simulink model "tanque_feedforward"  (Simulink 8.3)
settings: Solver=ode45  StartTime=0.0  StopTime=600  RelTol=1e-3
settings Model: Creator=Lideq2  LastModifiedBy=marcio
settings OptimizationCC: ExpressionDepthLimit=2147483647  InitFltsAndDblsToZero=on
settings DebuggingCC: SaveWithParameterizedLinksMsg=none  MultiTaskDSMMsg=warning  MultiTaskCondExecSysMsg=none  FcnCallInpInsideContextMsg=UseLocalSettings
settings RTWCC: IncludeERTFirstTime=on
settings GRTTargetCC: TargetFcnLib=ansi_tfl_tmw.mat

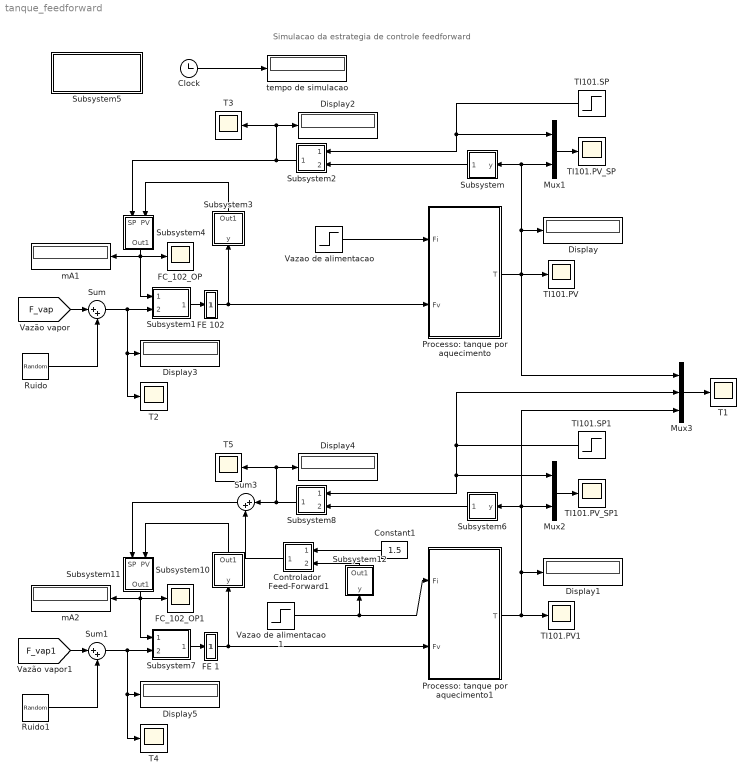
== system tanque_feedforward ==
  note: Simulacao da estrategia de controle feedforward
  Clock : Clock
  Constant1 : Constant  Value=1.5
  Controlador  Feed-Forward1 : Subsystem
      mask Display:
      | disp('AX\n411')
      | 
      | plot([   -5.0000   -4.9000   -4.8000   -4.7000    -4.6000   -4.5000   -4.4000   -4.3000  -4.2000   -4.1000   -4.0000   -3.9000    -3.8000   -3.7000   -3.6000   -3.5000    -3.4000   -3.3000   -3.2000   -3.1000    -3.0000   -2.9000   -2.8000   -2.7000    -2.6000   -2.5000   -2.4000   -2.3000    -2.2000   -2.1000   -2.0000   -1.9000    -1.8000   -1.7000   -1.6000   -1.5000    -1.4000   -1.3000   -1.2000   -1.1000    -1.0000   -0.9000   -0.8000   -0.7000    -0.6000   -0.5000   -0.4000   -0.3000    -0.2000   -0.1000         0    0.1000     0.2000    0.3000    0.4000    0.5000     0.6000    0.7000    0.8000    0.9000     1.0000    1.1000    1.2000    1.3000     1.4000    1.5000    1.6000    1.7000     1.8000    1.9000    2.0000    2.1000     2.2000    2.3000    2.4000    2.5000     2.6000    2.7000    2.8000    2.9000     3.0000    3.1000    3.2000    3.3000     3.4000    3.5000    3.6000    3.7000     3.8000    3.9000    4.0000    4.1000     4.2000    4.3000    4.4000    4.5000     4.6000    4.7000    4.8000    4.9000     5.0000], [0    0.9950    1.4000    1.7059     1.9596    2.1794    2.3749    2.5515    2.7129    2.8618    3.0000    3.1289    3.2496    3.3630    3.4699    3.5707     3.6661    3.7563    3.8419    3.9230    4.0000    4.0731    4.1425    4.2083    4.2708    4.3301    4.3863    4.4396    4.4900    4.5376    4.5826    4.6249    4.6648    4.7021    4.7371    4.7697    4.8000    4.8280    4.8539    4.8775     4.8990    4.9183    4.9356    4.9508    4.9639    4.9749    4.9840    4.9910    4.9960    4.9990    5.0000    4.9990    4.9960    4.9910    4.9840    4.9749    4.9639    4.9508    4.9356    4.9183    4.8990    4.8775    4.8539    4.8280    4.8000    4.7697    4.7371    4.7021    4.6648    4.6249    4.5826    4.5376    4.4900    4.4396    4.3863    4.3301    4.2708    4.2083    4.1425    4.0731    4.0000    3.9230    3.8419    3.7563    3.6661    3.5707    3.4699    3.3630    3.2496    3.1289    3.0000    2.8618    2.7129    2.5515    2.3749    2.1794     1.9596    1.7059    1.4000    0.9950         0], [   -5.0000   -4.9000   -4.8000   -4.7000    -4.6000   -4.5000   -4.4000   -4.3000  -4.2000   -4.1000   -4.0000   -3.9000    -3.8000   -3.7000   -3.6000   -3.5000    -3.4000   -3.3000   -3.2000   -3.1000    -3.0000   -2.9000   -2.8000   -2.7000    -2.6000   -2.5000   -2.4000   -2.3000    -2.2000   -2.1000   -2.0000   -1.9000    -1.8000   -1.7000   -1.6000   -1.5000    -1.4000   -1.3000   -1.2000   -1.1000    -1.0000   -0.9000   -0.8000   -0.7000    -0.6000   -0.5000   -0.4000   -0.3000    -0.2000   -0.1000         0    0.1000     0.2000    0.3000    0.4000    0.5000     0.6000    0.7000    0.8000    0.9000     1.0000    1.1000    1.2000    1.3000     1.4000    1.5000    1.6000    1.7000     1.8000    1.9000    2.0000    2.1000     2.2000    2.3000    2.4000    2.5000     2.6000    2.7000    2.8000    2.9000     3.0000    3.1000    3.2000    3.3000     3.4000    3.5000    3.6000    3.7000     3.8000    3.9000    4.0000    4.1000     4.2000    4.3000    4.4000    4.5000     4.6000    4.7000    4.8000    4.9000     5.0000], -[0    0.9950    1.4000    1.7059     1.9596    2.1794    2.3749    2.5515    2.7129    2.8618    3.0000    3.1289    3.2496    3.3630    3.4699    3.5707     3.6661    3.7563    3.8419    3.9230    4.0000    4.0731    4.1425    4.2083    4.2708    4.3301    4.3863    4.4396    4.4900    4.5376    4.5826    4.6249    4.6648    4.7021    4.7371    4.7697    4.8000    4.8280    4.8539    4.8775     4.8990    4.9183    4.9356    4.9508    4.9639    4.9749    4.9840    4.9910    4.9960    4.9990    5.0000    4.9990    4.9960    4.9910    4.9840    4.9749    4.9639    4.9508    4.9356    4.9183    4.8990    4.8775    4.8539    4.8280    4.8000    4.7697    4.7371    4.7021    4.6648    4.6249    4.5826    4.5376    4.4900    4.4396    4.3863    4.3301    4.2708    4.2083    4.1425    4.0731    4.0000    3.9230    3.8419    3.7563    3.6661    3.5707    3.4699    3.3630    3.2496    3.1289    3.0000    2.8618    2.7129    2.5515    2.3749    2.1794     1.9596    1.7059    1.4000    0.9950         0])
  Display{,1..5} (6 alike) : Display
  FC_102_OP : Scope
      settings: SaveName=FC_102_OP
  FC_102_OP1 : Scope
      settings: SaveName=FC_102_OP1
  FE 1 : Subsystem
      mask Display: plot(-1*ones(1,21),[-2:0.2:2],zeros(1,11),[-1:0.2:1],1*ones(1,21),[-2:0.2:2])
  FE 102 : Subsystem
      mask Display: plot(-1*ones(1,21),[-2:0.2:2],zeros(1,11),[-1:0.2:1],1*ones(1,21),[-2:0.2:2])
  Mux1 : Mux  Inputs=2
  Mux2 : Mux  Inputs=2
  Mux3 : Mux  Inputs=3
  Processo: tanque por aquecimento : Subsystem  mask(Teste){Fi=1.5, Fv=0.4, T=57}
      mask prompts: Fi "Estado estacionário da vazão de alimentação do tanque [=] t/min"; Fv "Estado estacionário da vazão de vapor do tanque [=] t/min"; T "Temperatura de saída do tanque"
      mask help: Testando descrição
      mask init:
      | x = -1:.1:1;
      | y1 =  x;
      | y2 = -x;
      | 
      | x1 = zeros(1,3);
      | y3 = [0 1 7];
      | 
      | y4 = -1:.1:1;
      | r = sqrt(2);
      | x2 = sqrt(r^2-y4.^2);
      | x3 = -sqrt(r^2-y4.^2);
      | 
      | xs = -sqrt(2)-.5:0.1:sqrt(2)+.5;
      | ys = sin(10000*xs)/3-sqrt(2)-.3;
      | 
      | y1t = y1 + 3;
      | y2t = y2 + 3;
      | 
      | y4t = 2:.1:4;
      | x2t =  sqrt(r^2-(y4t-3).^2);
      | x3t = -sqrt(r^2-(y4t-3).^2);
      mask Help: TESTANDO HELP
      mask Display:
      | plot(x,y1,x,y2,x1,y3,x2,y4,x3,y4,xs,ys)
      | plot(x,y1t,x,y2t,x2t,y4t,x3t,y4t)
      | plot(sqrt(2)+0.5,0,-sqrt(2)-0.5,0)
  Processo: tanque por aquecimento1 : Subsystem  mask(Teste){Fi=1.5, Fv=0.4, T=57}
      mask prompts: Fi "Estado estacionário da vazão de alimentação do tanque [=] t/min"; Fv "Estado estacionário da vazão de vapor do tanque [=] t/min"; T "Temperatura de saída do tanque"
      mask help: Testando descrição
      mask init: same as tanque_feedforward/Processo: tanque por aquecimento
      mask Help: TESTANDO HELP
      mask Display:
      | plot(x,y1,x,y2,x1,y3,x2,y4,x3,y4,xs,ys)
      | plot(x,y1t,x,y2t,x2t,y4t,x3t,y4t)
      | plot(sqrt(2)+0.5,0,-sqrt(2)-0.5,0)
  Ruido : RandomNumber  Variance=0.001  SampleTime=0
  Ruido1 : RandomNumber  Variance=0.001  SampleTime=0
  Subsystem : Subsystem  mask(Transmissor){ymax=100, ymin=0}
      mask prompts: ymax "Valor máximo da variavel"; ymin "Valor minimo da variavel"
      mask init:
      | x = -1:.1:1;
      | r = 1;
      | y1 = sqrt(r^2 - x.^2);
      | y2 = -sqrt(r^2 - x.^2);
      mask Display:
      | disp('TT')
      | plot(x,y1,x,y2)
  Subsystem1 : Subsystem  mask{Fmax=0.8, Fmin=0, talv=0.05}
      mask prompts: Fmax "Vazão máxima da valvula"; Fmin "Vazão minima da valvula"; talv "Dinâmica da valvula"
      mask init:
      | x= -1:.1:1;
      | 
      | y1=x;
      | y2=-x;
      | 
      | x1=[1,1];
      | y3=[1,-1];
      | x2=[-1,-1];
      | 
      | x3=[0,0,0];
      | y4=[0,1,2];
      | 
      | r=0.8;
      | x6= -r:.1:r;
      | y6 = sqrt(r^2-x6.^2)+2;
      | 
      | x5= [-r,r];
      | y5=[2,2];
      mask Display:
      | plot(x,y1,x,y2,x1,y3,x2,y3,x3,y4,x5,y5)
      | plot(x6,y6)
  Subsystem10 : Subsystem  mask(Transmissor){ymax=0.4*2, ymin=0}
      mask prompts: ymax "Valor máximo da variavel"; ymin "Valor minimo da variavel"
      mask init:
      | x = -1:.1:1;
      | r = 1;
      | y1 = sqrt(r^2 - x.^2);
      | y2 = -sqrt(r^2 - x.^2);
      mask Display:
      | disp('FT')
      | plot(x,y1,x,y2)
  Subsystem11 : Subsystem  mask(Controlador){AC=1, kc=3, tal_i=0.05, tal_d=0, BIAS=50, MODO=1}
      mask prompts: AC "Ação do controlador"; kc "Ganho do controlador"; tal_i "Constante de tempo integral"; tal_d "Constante de tempo derivativa"; BIAS "Posição da valvula em manual"; MODO "Modo de controle"
      mask init:
      | x = -1:.1:1;
      | r = 1;
      | y1 = sqrt(r^2 - x.^2);
      | y2 = -sqrt(r^2 - x.^2);
      mask Display:
      | disp('FC')
      | plot(x,y1,x,y2)
  Subsystem12 : Subsystem  mask(Transmissor){ymax=1.5*2, ymin=0}
      mask prompts: ymax "Valor máximo da variavel"; ymin "Valor minimo da variavel"
      mask init:
      | x = -1:.1:1;
      | r = 1;
      | y1 = sqrt(r^2 - x.^2);
      | y2 = -sqrt(r^2 - x.^2);
      mask Display:
      | disp('FT')
      | plot(x,y1,x,y2)
  Subsystem2 : Subsystem  mask(Controlador){AC=1, kc=2.4, tal_i=4.32, tal_d=0.05, BIAS=50, MODO=1}
      mask prompts: AC "Ação do controlador"; kc "Ganho do controlador"; tal_i "Constante de tempo integral"; tal_d "Constante de tempo derivativa"; BIAS "Posição da valvula em manual"; MODO "Modo de controle"
      mask init:
      | x = -1:.1:1;
      | r = 1;
      | y1 = sqrt(r^2 - x.^2);
      | y2 = -sqrt(r^2 - x.^2);
      mask Display:
      | disp('TC')
      | plot(x,y1,x,y2)
  Subsystem3 : Subsystem  mask(Transmissor){ymax=0.4*2, ymin=0}
      mask prompts: ymax "Valor máximo da variavel"; ymin "Valor minimo da variavel"
      mask init:
      | x = -1:.1:1;
      | r = 1;
      | y1 = sqrt(r^2 - x.^2);
      | y2 = -sqrt(r^2 - x.^2);
      mask Display:
      | disp('FT')
      | plot(x,y1,x,y2)
  Subsystem4 : Subsystem  mask(Controlador){AC=1, kc=3, tal_i=0.05, tal_d=0, BIAS=50, MODO=1}
      mask prompts: AC "Ação do controlador"; kc "Ganho do controlador"; tal_i "Constante de tempo integral"; tal_d "Constante de tempo derivativa"; BIAS "Posição da valvula em manual"; MODO "Modo de controle"
      mask init:
      | x = -1:.1:1;
      | r = 1;
      | y1 = sqrt(r^2 - x.^2);
      | y2 = -sqrt(r^2 - x.^2);
      mask Display:
      | disp('FC')
      | plot(x,y1,x,y2)
  Subsystem5 : Subsystem
      settings: OpenFcn=save tanque
      mask Display: disp('Salvar \n dados')
  Subsystem6 : Subsystem  mask(Transmissor){ymax=100, ymin=0}
      mask prompts: ymax "Valor máximo da variavel"; ymin "Valor minimo da variavel"
      mask init:
      | x = -1:.1:1;
      | r = 1;
      | y1 = sqrt(r^2 - x.^2);
      | y2 = -sqrt(r^2 - x.^2);
      mask Display:
      | disp('TT')
      | plot(x,y1,x,y2)
  Subsystem7 : Subsystem  mask{Fmax=0.8, Fmin=0, talv=0.05}
      mask prompts: Fmax "Vazão máxima da valvula"; Fmin "Vazão minima da valvula"; talv "Dinâmica da valvula"
      mask init:
      | x= -1:.1:1;
      | 
      | y1=x;
      | y2=-x;
      | 
      | x1=[1,1];
      | y3=[1,-1];
      | x2=[-1,-1];
      | 
      | x3=[0,0,0];
      | y4=[0,1,2];
      | 
      | r=0.8;
      | x6= -r:.1:r;
      | y6 = sqrt(r^2-x6.^2)+2;
      | 
      | x5= [-r,r];
      | y5=[2,2];
      mask Display:
      | plot(x,y1,x,y2,x1,y3,x2,y3,x3,y4,x5,y5)
      | plot(x6,y6)
  Subsystem8 : Subsystem  mask(Controlador){AC=1, kc=2.4, tal_i=4.32, tal_d=0.05, BIAS=50, MODO=1}
      mask prompts: AC "Ação do controlador"; kc "Ganho do controlador"; tal_i "Constante de tempo integral"; tal_d "Constante de tempo derivativa"; BIAS "Posição da valvula em manual"; MODO "Modo de controle"
      mask init:
      | x = -1:.1:1;
      | r = 1;
      | y1 = sqrt(r^2 - x.^2);
      | y2 = -sqrt(r^2 - x.^2);
      mask Display:
      | disp('TC')
      | plot(x,y1,x,y2)
  Sum : Sum  Inputs=|++
  Sum1 : Sum  Inputs=|++
  Sum3 : Sum  Inputs=|++
  T{1..5} (5 alike) : Scope
      T1 settings: SaveName=ScopeData9
      T2 settings: SaveName=ScopeData2
      T3 settings: SaveName=ScopeData4
      T4 settings: SaveName=ScopeData5
      T5 settings: SaveName=ScopeData6
  TI101.PV : Scope
  TI101.PV1 : Scope
      settings: SaveName=ScopeData7
  TI101.PV_SP : Scope
  TI101.PV_SP1 : Scope
      settings: SaveName=ScopeData8
  TI101.SP : Step  Time=50  Before=57  After=57*1.1  SampleTime=0
  TI101.SP1 : Step  Time=50  Before=57  After=57*1.1  SampleTime=0
  Vazao de alimentacao : Step  Time=300  Before=1.5  After=1.5*1.35  SampleTime=0
  Vazao de alimentacao1 : Step  Time=300  Before=1.5  After=1.5*1.35  SampleTime=0
  mA1 : Display
  mA2 : Display
  tempo de simulacao : Display
  wires:
  Processo: tanque por aquecimento/1(T) -> TI101.PV/1, Display/1, Subsystem/1(y), Mux1/2, Mux3/1
  Vazao de alimentacao/1 -> Processo: tanque por aquecimento/1(Fi)
  Subsystem/1(Out1) -> Subsystem2/2(PV)
  Subsystem2/1(Out1) -> Display2/1, T3/1, Subsystem4/1(SP)
  Mux1/1 -> TI101.PV_SP/1
  TI101.SP/1 -> Subsystem2/1(SP), Mux1/1
  Sum/1 -> Subsystem1/2(In2), Display3/1, T2/1
  [F_vap] -> Sum/1
  Ruido/1 -> Sum/2
  Subsystem3/1(Out1) -> Subsystem4/2(PV)
  Subsystem1/1(Out2) -> FE 102/1(In1)
  FE 102/1(Out2) -> Processo: tanque por aquecimento/2(Fv), Subsystem3/1(y)
  Subsystem4/1(Out1) -> FC_102_OP/1, mA1/1, Subsystem1/1(In1)
  Clock/1 -> tempo de simulacao/1
  Mux3/1 -> T1/1
  Processo: tanque por aquecimento1/1(T) -> Mux2/2, Subsystem6/1(y), Mux3/3, Display1/1, TI101.PV1/1
  Vazao de alimentacao1/1 -> Processo: tanque por aquecimento1/1(Fi), Subsystem12/1(y)
  Subsystem6/1(Out1) -> Subsystem8/2(PV)
  Subsystem8/1(Out1) -> Sum3/1, T5/1, Display4/1
  Mux2/1 -> TI101.PV_SP1/1
  TI101.SP1/1 -> Mux2/1, Subsystem8/1(SP), Mux3/2
  Sum1/1 -> T4/1, Display5/1, Subsystem7/2(In2)
  [F_vap1] -> Sum1/1
  Ruido1/1 -> Sum1/2
  Subsystem10/1(Out1) -> Subsystem11/2(PV)
  Subsystem7/1(Out2) -> FE 1/1(In1)
  FE 1/1(Out2) -> Subsystem10/1(y), Processo: tanque por aquecimento1/2(Fv)
  Subsystem11/1(Out1) -> Subsystem7/1(In1), mA2/1, FC_102_OP1/1
  Constant1/1 -> Controlador  Feed-Forward1/1(Set-Point do distúrbio externo)
  Sum3/1 -> Subsystem11/1(SP)
  Controlador  Feed-Forward1/1(Out1) -> Sum3/2
  Subsystem12/1(Out1) -> Controlador  Feed-Forward1/2(Sinal do distúrbio externo)

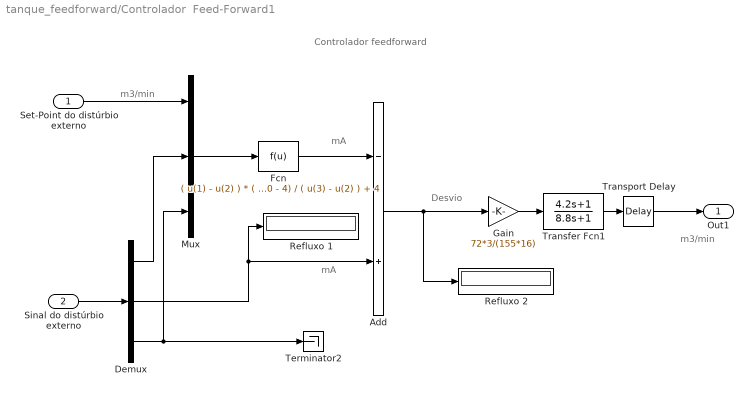
== system tanque_feedforward/Controlador  Feed-Forward1 ==
  note: m3/min
  note: Desvio
  note: mA
  note: mA
  note: m3/min
  note: Controlador feedforward
  Set-Point do distúrbio externo : Inport
  Sinal do distúrbio externo : Inport  Port=2
  Add : Sum  Inputs=-+
  Demux : Demux  Outputs=3
  Fcn : Fcn  Expr=( u(1) - u(2) ) * ( 20 - 4) / ( u(3) - u(2) ) + 4
  Gain : Gain  Gain=72*3/(155*16)
  Mux : Mux  Inputs=3
  Refluxo 1 : Display
  Refluxo 2 : Display
  Terminator2 : Terminator
  Transfer Fcn1 : TransferFcn  Numerator=[4.2 1]  Denominator=[8.8 1]
  Transport Delay : TransportDelay  DelayTime=2
  Out1 : Outport
  wires:
  Demux/1 -> Mux/2
  Demux/2 -> Refluxo 1/1, Add/2
  Transport Delay/1 -> Out1/1
  Add/1 -> Refluxo 2/1, Gain/1
  Fcn/1 -> Add/1
  Mux/1 -> Fcn/1
  Set-Point do distúrbio externo/1 -> Mux/1
  Demux/3 -> Mux/3, Terminator2/1
  Sinal do distúrbio externo/1 -> Demux/1
  Transfer Fcn1/1 -> Transport Delay/1
  Gain/1 -> Transfer Fcn1/1

== system tanque_feedforward/FE 1 ==
  note: Placa de orifício
  In1 : Inport
  Out2 : Outport
  wires:
  In1/1 -> Out2/1

== system tanque_feedforward/FE 102 ==
  note: Placa de orifício
  In1 : Inport
  Out2 : Outport
  wires:
  In1/1 -> Out2/1

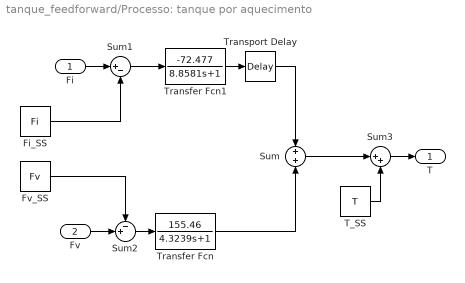
== system tanque_feedforward/Processo: tanque por aquecimento ==
  Fi : Inport
  Fv : Inport  Port=2
  Fi_SS : Constant  Value=Fi
  Fv_SS : Constant  Value=Fv
  Sum : Sum  Inputs=+|+
  Sum1 : Sum  Inputs=|+-
  Sum2 : Sum  Inputs=-+|
  Sum3 : Sum  Inputs=|++
  T_SS : Constant  Value=T
  Transfer Fcn : TransferFcn  Numerator=[155.46]  Denominator=[4.3239 1]
  Transfer Fcn1 : TransferFcn  Numerator=[-72.477]  Denominator=[8.8581 1]
  Transport Delay : TransportDelay  DelayTime=2
  T : Outport
  wires:
  Sum/1 -> Sum3/1
  T_SS/1 -> Sum3/2
  Fi_SS/1 -> Sum1/2
  Fv_SS/1 -> Sum2/1
  Fi/1 -> Sum1/1
  Sum3/1 -> T/1
  Fv/1 -> Sum2/2
  Sum1/1 -> Transfer Fcn1/1
  Sum2/1 -> Transfer Fcn/1
  Transfer Fcn1/1 -> Transport Delay/1
  Transport Delay/1 -> Sum/1
  Transfer Fcn/1 -> Sum/2

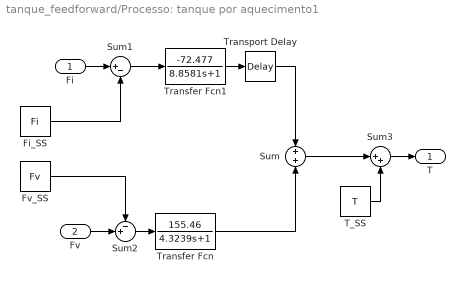
== system tanque_feedforward/Processo: tanque por aquecimento1 ==
  Fi : Inport
  Fv : Inport  Port=2
  Fi_SS : Constant  Value=Fi
  Fv_SS : Constant  Value=Fv
  Sum : Sum  Inputs=+|+
  Sum1 : Sum  Inputs=|+-
  Sum2 : Sum  Inputs=-+|
  Sum3 : Sum  Inputs=|++
  T_SS : Constant  Value=T
  Transfer Fcn : TransferFcn  Numerator=[155.46]  Denominator=[4.3239 1]
  Transfer Fcn1 : TransferFcn  Numerator=[-72.477]  Denominator=[8.8581 1]
  Transport Delay : TransportDelay  DelayTime=2
  T : Outport
  wires:
  Transfer Fcn/1 -> Sum/2
  Transport Delay/1 -> Sum/1
  Transfer Fcn1/1 -> Transport Delay/1
  Sum2/1 -> Transfer Fcn/1
  Sum1/1 -> Transfer Fcn1/1
  Fv/1 -> Sum2/2
  Sum3/1 -> T/1
  Fi/1 -> Sum1/1
  Fv_SS/1 -> Sum2/1
  Fi_SS/1 -> Sum1/2
  T_SS/1 -> Sum3/2
  Sum/1 -> Sum3/1

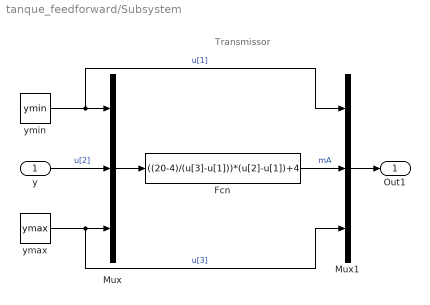
== system tanque_feedforward/Subsystem ==
  note: Transmissor
  y : Inport
  Fcn : Fcn  Expr=((20-4)/(u[3]-u[1]))*(u[2]-u[1])+4
  Mux : Mux  Inputs=3
  Mux1 : Mux  Inputs=3
  ymax : Constant  Value=ymax
  ymin : Constant  Value=ymin
  Out1 : Outport
  wires:
  ymin/1 -> Mux/1, Mux1/1  "u[1]"
  y/1 -> Mux/2  "u[2]"
  ymax/1 -> Mux/3, Mux1/3  "u[3]"
  Mux/1 -> Fcn/1
  Fcn/1 -> Mux1/2  "mA"
  Mux1/1 -> Out1/1

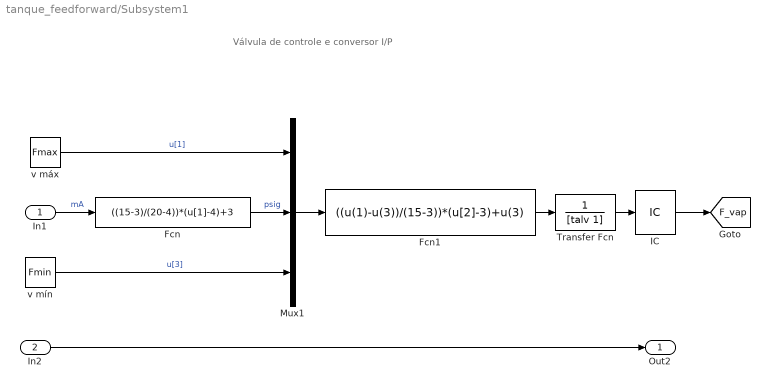
== system tanque_feedforward/Subsystem1 ==
  note: Válvula de controle e conversor I/P
  In1 : Inport
  In2 : Inport  Port=2
  Fcn : Fcn  Expr=((15-3)/(20-4))*(u[1]-4)+3
  Fcn1 : Fcn  Expr=((u(1)-u(3))/(15-3))*(u[2]-3)+u(3)
  IC : InitialCondition  Value=0.4
  Mux1 : Mux  Inputs=3
  Transfer Fcn : TransferFcn  Denominator=[talv 1]
  v máx : Constant  Value=Fmax
  v mín : Constant  Value=Fmin
  Out2 : Outport
  tag scope: F_vap=global
  wires:
  Fcn/1 -> Mux1/2  "psig"
  In1/1 -> Fcn/1  "mA"
  Mux1/1 -> Fcn1/1
  v máx/1 -> Mux1/1  "u[1]"
  v mín/1 -> Mux1/3  "u[3]"
  In2/1 -> Out2/1
  Fcn1/1 -> Transfer Fcn/1
  IC/1 -> [F_vap]
  Transfer Fcn/1 -> IC/1

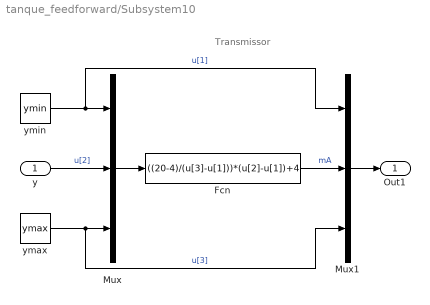
== system tanque_feedforward/Subsystem10 ==
  note: Transmissor
  y : Inport
  Fcn : Fcn  Expr=((20-4)/(u[3]-u[1]))*(u[2]-u[1])+4
  Mux : Mux  Inputs=3
  Mux1 : Mux  Inputs=3
  ymax : Constant  Value=ymax
  ymin : Constant  Value=ymin
  Out1 : Outport
  wires:
  ymin/1 -> Mux/1, Mux1/1  "u[1]"
  y/1 -> Mux/2  "u[2]"
  ymax/1 -> Mux/3, Mux1/3  "u[3]"
  Mux/1 -> Fcn/1
  Fcn/1 -> Mux1/2  "mA"
  Mux1/1 -> Out1/1

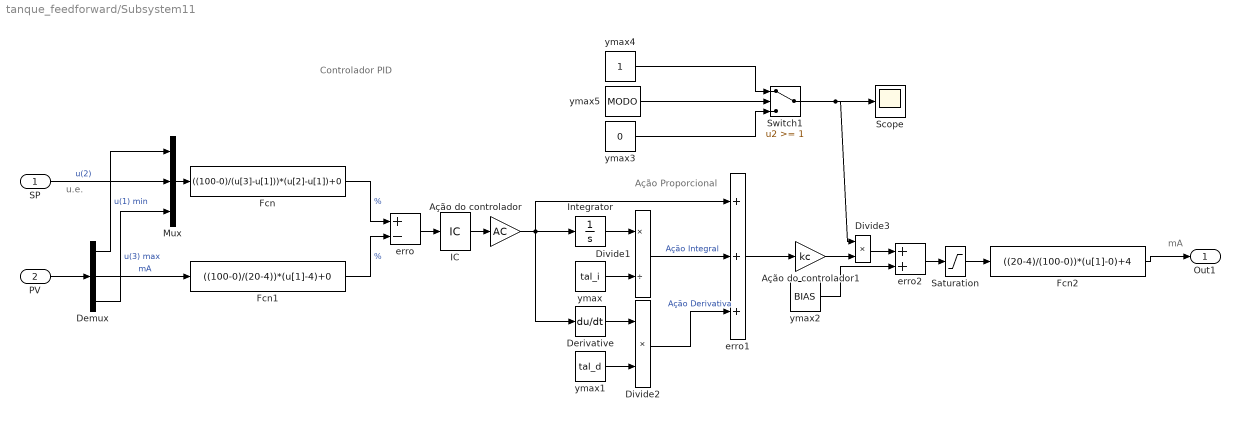
== system tanque_feedforward/Subsystem11 ==
  note: Controlador PID
  note: u.e.
  note: Ação Proporcional
  note: mA
  SP : Inport
  PV : Inport  Port=2
  Ação do controlador : Gain  Gain=AC
  Ação do controlador1 : Gain  Gain=kc
  Demux : Demux  Outputs=3
  Derivative : Derivative
  Divide1 : Product  Inputs=*/
  Divide2 : Product
  Divide3 : Product
  Fcn : Fcn  Expr=((100-0)/(u[3]-u[1]))*(u[2]-u[1])+0
  Fcn1 : Fcn  Expr=((100-0)/(20-4))*(u[1]-4)+0
  Fcn2 : Fcn  Expr=((20-4)/(100-0))*(u[1]-0)+4
  IC : InitialCondition  Value=0
  Integrator : Integrator
  Mux : Mux  Inputs=3
  Saturation : Saturate  UpperLimit=100  LowerLimit=0
  Scope : Scope
      settings: SaveName=ScopeData3
  Switch1 : Switch  Threshold=1
  erro : Sum  Inputs=+-
  erro1 : Sum  Inputs=+++
  erro2 : Sum
  ymax : Constant  Value=tal_i
  ymax1 : Constant  Value=tal_d
  ymax2 : Constant  Value=BIAS
  ymax3 : Constant  Value=0
  ymax4 : Constant
  ymax5 : Constant  Value=MODO
  Out1 : Outport
  wires:
  PV/1 -> Demux/1
  SP/1 -> Mux/2  "u(2)"
  Demux/1 -> Mux/1  "u(1) min"
  Demux/3 -> Mux/3  "u(3) max"
  Mux/1 -> Fcn/1
  Demux/2 -> Fcn1/1  "mA"
  Fcn/1 -> erro/1  "%"
  Fcn1/1 -> erro/2  "%"
  erro/1 -> IC/1
  Ação do controlador/1 -> Integrator/1, erro1/1, Derivative/1
  Integrator/1 -> Divide1/1
  ymax/1 -> Divide1/2
  Divide1/1 -> erro1/2  "Ação Integral"
  Derivative/1 -> Divide2/1
  ymax1/1 -> Divide2/2
  Divide2/1 -> erro1/3  "Ação Derivativa"
  erro1/1 -> Ação do controlador1/1
  ymax2/1 -> erro2/2
  erro2/1 -> Saturation/1
  ymax5/1 -> Switch1/2
  ymax4/1 -> Switch1/1
  ymax3/1 -> Switch1/3
  Divide3/1 -> erro2/1
  Ação do controlador1/1 -> Divide3/2
  Switch1/1 -> Divide3/1, Scope/1
  Saturation/1 -> Fcn2/1
  Fcn2/1 -> Out1/1
  IC/1 -> Ação do controlador/1

== system tanque_feedforward/Subsystem12 ==
  note: Transmissor
  y : Inport
  Fcn : Fcn  Expr=((20-4)/(u[3]-u[1]))*(u[2]-u[1])+4
  Mux : Mux  Inputs=3
  Mux1 : Mux  Inputs=3
  ymax : Constant  Value=ymax
  ymin : Constant  Value=ymin
  Out1 : Outport
  wires:
  Mux1/1 -> Out1/1
  Fcn/1 -> Mux1/2  "mA"
  Mux/1 -> Fcn/1
  ymax/1 -> Mux1/3, Mux/3  "u[3]"
  y/1 -> Mux/2  "u[2]"
  ymin/1 -> Mux1/1, Mux/1  "u[1]"

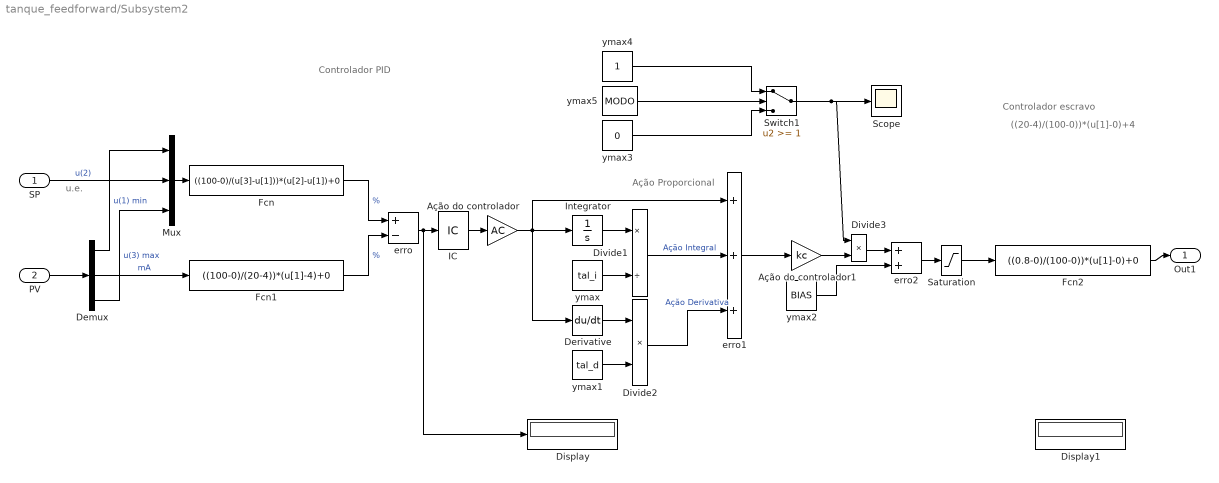
== system tanque_feedforward/Subsystem2 ==
  note: Controlador PID
  note: u.e.
  note: Ação Proporcional
  note: ((20-4)/(100-0))*(u[1]-0)+4
  note: Controlador escravo
  SP : Inport
  PV : Inport  Port=2
  Ação do controlador : Gain  Gain=AC
  Ação do controlador1 : Gain  Gain=kc
  Demux : Demux  Outputs=3
  Derivative : Derivative
  Display : Display
  Display1 : Display
  Divide1 : Product  Inputs=*/
  Divide2 : Product
  Divide3 : Product
  Fcn : Fcn  Expr=((100-0)/(u[3]-u[1]))*(u[2]-u[1])+0
  Fcn1 : Fcn  Expr=((100-0)/(20-4))*(u[1]-4)+0
  Fcn2 : Fcn  Expr=((0.8-0)/(100-0))*(u[1]-0)+0
  IC : InitialCondition  Value=0
  Integrator : Integrator
  Mux : Mux  Inputs=3
  Saturation : Saturate  UpperLimit=100  LowerLimit=0
  Scope : Scope
      settings: SaveName=ScopeData3
  Switch1 : Switch  Threshold=1
  erro : Sum  Inputs=+-
  erro1 : Sum  Inputs=+++
  erro2 : Sum
  ymax : Constant  Value=tal_i
  ymax1 : Constant  Value=tal_d
  ymax2 : Constant  Value=BIAS
  ymax3 : Constant  Value=0
  ymax4 : Constant
  ymax5 : Constant  Value=MODO
  Out1 : Outport
  wires:
  PV/1 -> Demux/1
  SP/1 -> Mux/2  "u(2)"
  Demux/1 -> Mux/1  "u(1) min"
  Demux/3 -> Mux/3  "u(3) max"
  Mux/1 -> Fcn/1
  Demux/2 -> Fcn1/1  "mA"
  Fcn/1 -> erro/1  "%"
  Fcn1/1 -> erro/2  "%"
  erro/1 -> IC/1, Display/1
  Ação do controlador/1 -> Integrator/1, erro1/1, Derivative/1
  Integrator/1 -> Divide1/1
  ymax/1 -> Divide1/2
  Divide1/1 -> erro1/2  "Ação Integral"
  Derivative/1 -> Divide2/1
  ymax1/1 -> Divide2/2
  Divide2/1 -> erro1/3  "Ação Derivativa"
  erro1/1 -> Ação do controlador1/1
  ymax2/1 -> erro2/2
  erro2/1 -> Saturation/1
  ymax5/1 -> Switch1/2
  ymax4/1 -> Switch1/1
  ymax3/1 -> Switch1/3
  Divide3/1 -> erro2/1
  Ação do controlador1/1 -> Divide3/2
  Switch1/1 -> Divide3/1, Scope/1
  Fcn2/1 -> Out1/1
  IC/1 -> Ação do controlador/1
  Saturation/1 -> Fcn2/1

== system tanque_feedforward/Subsystem3 ==
  note: Transmissor
  y : Inport
  Fcn : Fcn  Expr=((20-4)/(u[3]-u[1]))*(u[2]-u[1])+4
  Mux : Mux  Inputs=3
  Mux1 : Mux  Inputs=3
  ymax : Constant  Value=ymax
  ymin : Constant  Value=ymin
  Out1 : Outport
  wires:
  Mux1/1 -> Out1/1
  Fcn/1 -> Mux1/2  "mA"
  Mux/1 -> Fcn/1
  ymax/1 -> Mux1/3, Mux/3  "u[3]"
  y/1 -> Mux/2  "u[2]"
  ymin/1 -> Mux1/1, Mux/1  "u[1]"

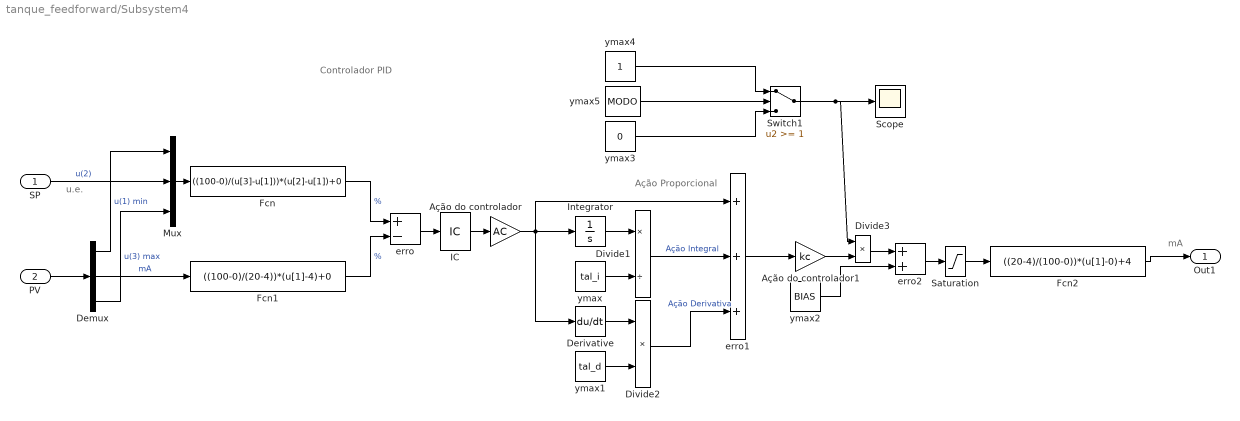
== system tanque_feedforward/Subsystem4 ==
  note: mA
  note: Ação Proporcional
  note: u.e.
  note: Controlador PID
  SP : Inport
  PV : Inport  Port=2
  Ação do controlador : Gain  Gain=AC
  Ação do controlador1 : Gain  Gain=kc
  Demux : Demux  Outputs=3
  Derivative : Derivative
  Divide1 : Product  Inputs=*/
  Divide2 : Product
  Divide3 : Product
  Fcn : Fcn  Expr=((100-0)/(u[3]-u[1]))*(u[2]-u[1])+0
  Fcn1 : Fcn  Expr=((100-0)/(20-4))*(u[1]-4)+0
  Fcn2 : Fcn  Expr=((20-4)/(100-0))*(u[1]-0)+4
  IC : InitialCondition  Value=0
  Integrator : Integrator
  Mux : Mux  Inputs=3
  Saturation : Saturate  UpperLimit=100  LowerLimit=0
  Scope : Scope
      settings: SaveName=ScopeData3
  Switch1 : Switch  Threshold=1
  erro : Sum  Inputs=+-
  erro1 : Sum  Inputs=+++
  erro2 : Sum
  ymax : Constant  Value=tal_i
  ymax1 : Constant  Value=tal_d
  ymax2 : Constant  Value=BIAS
  ymax3 : Constant  Value=0
  ymax4 : Constant
  ymax5 : Constant  Value=MODO
  Out1 : Outport
  wires:
  IC/1 -> Ação do controlador/1
  Fcn2/1 -> Out1/1
  Saturation/1 -> Fcn2/1
  Switch1/1 -> Scope/1, Divide3/1
  Ação do controlador1/1 -> Divide3/2
  Divide3/1 -> erro2/1
  ymax3/1 -> Switch1/3
  ymax4/1 -> Switch1/1
  ymax5/1 -> Switch1/2
  erro2/1 -> Saturation/1
  ymax2/1 -> erro2/2
  erro1/1 -> Ação do controlador1/1
  Divide2/1 -> erro1/3  "Ação Derivativa"
  ymax1/1 -> Divide2/2
  Derivative/1 -> Divide2/1
  Divide1/1 -> erro1/2  "Ação Integral"
  ymax/1 -> Divide1/2
  Integrator/1 -> Divide1/1
  Ação do controlador/1 -> Derivative/1, erro1/1, Integrator/1
  erro/1 -> IC/1
  Fcn1/1 -> erro/2  "%"
  Fcn/1 -> erro/1  "%"
  Demux/2 -> Fcn1/1  "mA"
  Mux/1 -> Fcn/1
  Demux/3 -> Mux/3  "u(3) max"
  Demux/1 -> Mux/1  "u(1) min"
  SP/1 -> Mux/2  "u(2)"
  PV/1 -> Demux/1

== system tanque_feedforward/Subsystem5 ==

== system tanque_feedforward/Subsystem6 ==
  note: Transmissor
  y : Inport
  Fcn : Fcn  Expr=((20-4)/(u[3]-u[1]))*(u[2]-u[1])+4
  Mux : Mux  Inputs=3
  Mux1 : Mux  Inputs=3
  ymax : Constant  Value=ymax
  ymin : Constant  Value=ymin
  Out1 : Outport
  wires:
  Mux1/1 -> Out1/1
  Fcn/1 -> Mux1/2  "mA"
  Mux/1 -> Fcn/1
  ymax/1 -> Mux1/3, Mux/3  "u[3]"
  y/1 -> Mux/2  "u[2]"
  ymin/1 -> Mux1/1, Mux/1  "u[1]"

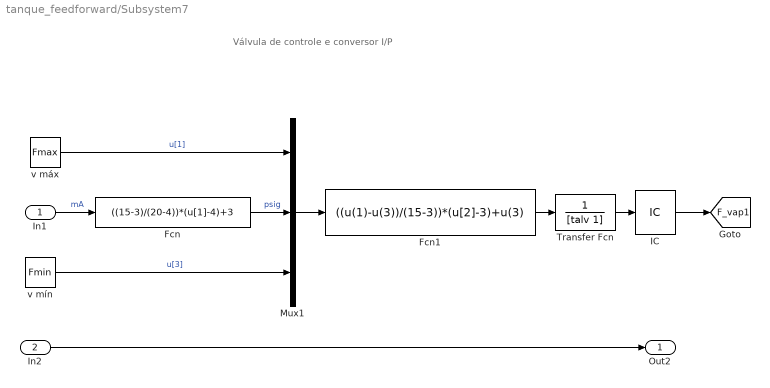
== system tanque_feedforward/Subsystem7 ==
  note: Válvula de controle e conversor I/P
  In1 : Inport
  In2 : Inport  Port=2
  Fcn : Fcn  Expr=((15-3)/(20-4))*(u[1]-4)+3
  Fcn1 : Fcn  Expr=((u(1)-u(3))/(15-3))*(u[2]-3)+u(3)
  IC : InitialCondition  Value=0.4
  Mux1 : Mux  Inputs=3
  Transfer Fcn : TransferFcn  Denominator=[talv 1]
  v máx : Constant  Value=Fmax
  v mín : Constant  Value=Fmin
  Out2 : Outport
  tag scope: F_vap1=global
  wires:
  Transfer Fcn/1 -> IC/1
  IC/1 -> [F_vap1]
  Fcn1/1 -> Transfer Fcn/1
  In2/1 -> Out2/1
  v mín/1 -> Mux1/3  "u[3]"
  v máx/1 -> Mux1/1  "u[1]"
  Mux1/1 -> Fcn1/1
  In1/1 -> Fcn/1  "mA"
  Fcn/1 -> Mux1/2  "psig"

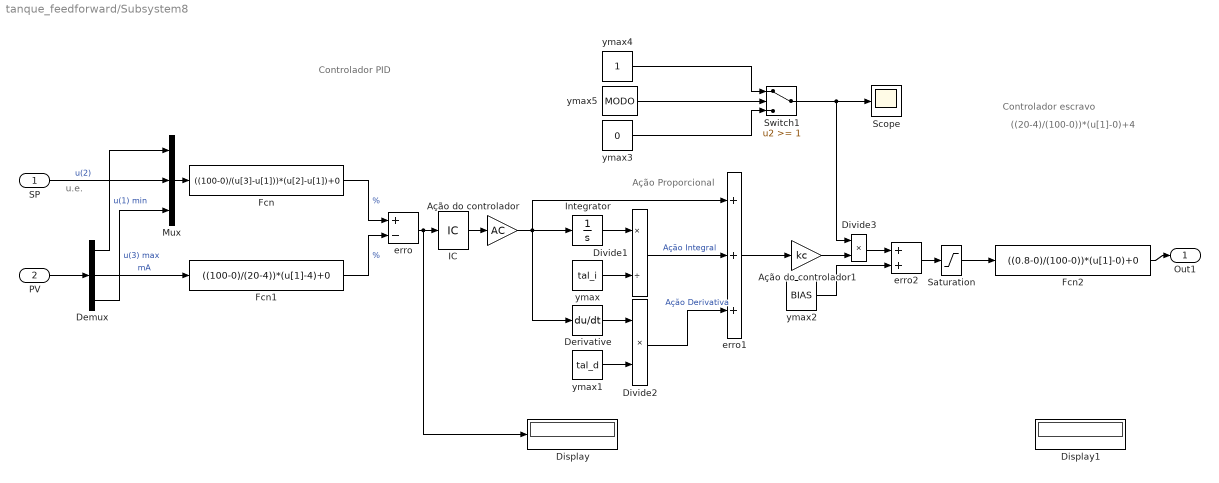
== system tanque_feedforward/Subsystem8 ==
  note: Controlador escravo
  note: ((20-4)/(100-0))*(u[1]-0)+4
  note: Ação Proporcional
  note: u.e.
  note: Controlador PID
  SP : Inport
  PV : Inport  Port=2
  Ação do controlador : Gain  Gain=AC
  Ação do controlador1 : Gain  Gain=kc
  Demux : Demux  Outputs=3
  Derivative : Derivative
  Display : Display
  Display1 : Display
  Divide1 : Product  Inputs=*/
  Divide2 : Product
  Divide3 : Product
  Fcn : Fcn  Expr=((100-0)/(u[3]-u[1]))*(u[2]-u[1])+0
  Fcn1 : Fcn  Expr=((100-0)/(20-4))*(u[1]-4)+0
  Fcn2 : Fcn  Expr=((0.8-0)/(100-0))*(u[1]-0)+0
  IC : InitialCondition  Value=0
  Integrator : Integrator
  Mux : Mux  Inputs=3
  Saturation : Saturate  UpperLimit=100  LowerLimit=0
  Scope : Scope
      settings: SaveName=ScopeData3
  Switch1 : Switch  Threshold=1
  erro : Sum  Inputs=+-
  erro1 : Sum  Inputs=+++
  erro2 : Sum
  ymax : Constant  Value=tal_i
  ymax1 : Constant  Value=tal_d
  ymax2 : Constant  Value=BIAS
  ymax3 : Constant  Value=0
  ymax4 : Constant
  ymax5 : Constant  Value=MODO
  Out1 : Outport
  wires:
  Saturation/1 -> Fcn2/1
  IC/1 -> Ação do controlador/1
  Fcn2/1 -> Out1/1
  Switch1/1 -> Scope/1, Divide3/1
  Ação do controlador1/1 -> Divide3/2
  Divide3/1 -> erro2/1
  ymax3/1 -> Switch1/3
  ymax4/1 -> Switch1/1
  ymax5/1 -> Switch1/2
  erro2/1 -> Saturation/1
  ymax2/1 -> erro2/2
  erro1/1 -> Ação do controlador1/1
  Divide2/1 -> erro1/3  "Ação Derivativa"
  ymax1/1 -> Divide2/2
  Derivative/1 -> Divide2/1
  Divide1/1 -> erro1/2  "Ação Integral"
  ymax/1 -> Divide1/2
  Integrator/1 -> Divide1/1
  Ação do controlador/1 -> Derivative/1, erro1/1, Integrator/1
  erro/1 -> Display/1, IC/1
  Fcn1/1 -> erro/2  "%"
  Fcn/1 -> erro/1  "%"
  Demux/2 -> Fcn1/1  "mA"
  Mux/1 -> Fcn/1
  Demux/3 -> Mux/3  "u(3) max"
  Demux/1 -> Mux/1  "u(1) min"
  SP/1 -> Mux/2  "u(2)"
  PV/1 -> Demux/1
